simulink model "ssc_cvt_test_harness"  (R2025a)
settings: Solver=VariableStepAuto  StartTime=0.0  StopTime=200  RelTol=1e-3
undefined symbols (not defined in the file or in its folder): HMPST
libraries: fl_lib x7, nesl_utility x5, sm_wheel_loader_lib x3, sdl_lib x2, simulink x1
Description:
  | CVT Test Harness
  | Copyright 2024-2025 The MathWorks, Inc.
settings Model: Creator=smiller  LastModifiedBy=smiller
settings SolverCC: MaxConsecutiveMinStep=5
settings SimscapeCC: SimscapeLogType=all

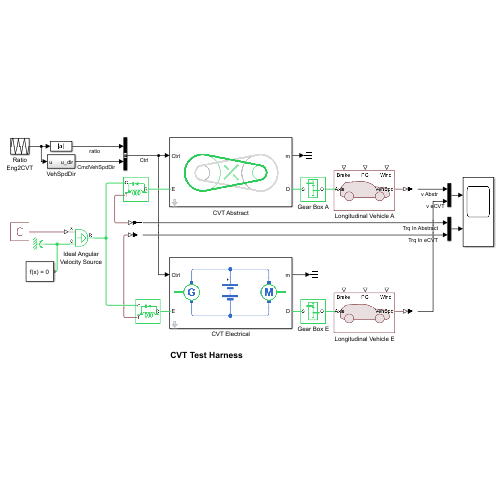
[thumbnail: Simulink's stored preview of the top-level diagram]
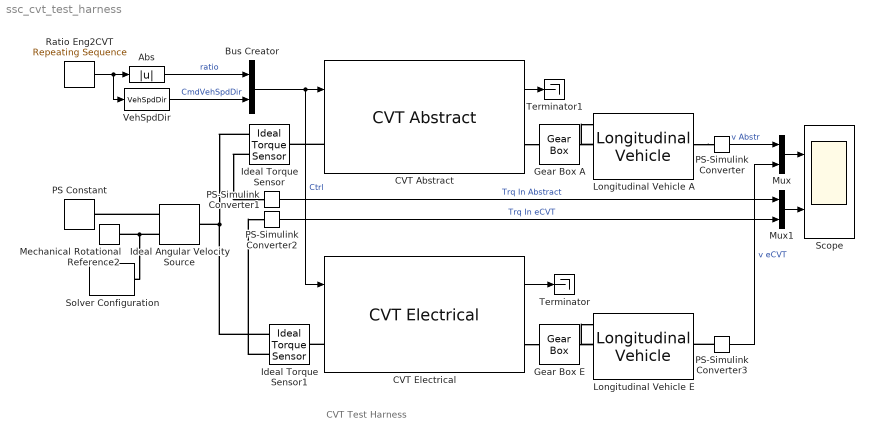
== system ssc_cvt_test_harness ==
  note: CVT Test Harness
  Abs : Abs  ZeroCross=off  SaturateOnIntegerOverflow=off
  Bus Creator : BusCreator  Inputs=2
  CVT Abstract : sm_wheel_loader_lib/CVT Abstract  dShaftE=HMPST.AbstractCVT.dInput  dShaftD=HMPST.AbstractCVT.dOutput  k=HMPST.AbstractCVT.kCompliance  d=HMPST.AbstractCVT.dCompliance
  CVT Electrical : sm_wheel_loader_lib/CVT Electrical  VariantControl=Electrical
  Gear Box A : fl_lib/Mechanical/Mechanisms/Gear Box  ratio=10  t_in_specify=off  t_in_priority=None  t_in=0 N*m  t_in_nominal_specify=off  t_in_nominal_value=1  t_in_nominal_unit=N*m  t_out_specify=off  t_out_priority=None  t_out=0 N*m  t_out_nominal_specify=off  t_out_nominal_value=1  t_out_nominal_unit=N*m
  Gear Box E : fl_lib/Mechanical/Mechanisms/Gear Box  ratio=10  t_in_specify=off  t_in_priority=None  t_in=0 N*m  t_in_nominal_specify=off  t_in_nominal_value=1  t_in_nominal_unit=N*m  t_out_specify=off  t_out_priority=None  t_out=0 N*m  t_out_nominal_specify=off  t_out_nominal_value=1  t_out_nominal_unit=N*m
  Ideal Angular Velocity Source : fl_lib/Mechanical/Mechanical Sources/Ideal Angular Velocity Source
  Ideal Torque Sensor : fl_lib/Mechanical/Mechanical Sensors/Ideal Torque Sensor
  Ideal Torque Sensor1 : fl_lib/Mechanical/Mechanical Sensors/Ideal Torque Sensor
  Longitudinal Vehicle A : sdl_lib/Tires & Vehicles/Longitudinal Vehicle  vehParamType=sdl.enum.VehicleParameterizationType.Regular  M_vehicle=3638 kg  R_tireroll=0.3 m  C_tireroll=0.0136  C_airdrag=0.31  A_front=2.3 m^2  A_rl=120 N  B_rl=1.8 N*s/m  C_rl=0.389 N*s^2/m^2  g=9.81 m/s^2  V_1=0.3 m/s  w_1=0.01 rad/s  ShowBrakeIn=true  ShowSlopeIn=true  SlopeInputType=sdl.enum.VehicleLongitudinalRoadSlopeInputType.GradePercent  ShowWindIn=true  ShowGOut=false  air_density=1.184 kg/m^3  V_x_specify=off  V_x_priority=High  V_x=0 m/s  V_x_nominal_specify=off  V_x_nominal_value=1  V_x_nominal_unit=m/s  trq_specify=off  trq_priority=None  trq=0 N*m  trq_nominal_specify=off  trq_nominal_value=1  trq_nominal_unit=N*m  w_specify=off  w_priority=None  w=0 rad/s  w_nominal_specify=off  w_nominal_value=1  w_nominal_unit=rad/s
      settings: InternalSimscapePortConfiguration="{\"Bottom\":[],\"Left\":[{\"id\":\"Axle\",\"label\":\"Axle\",\"type\":\"foundation.mechanical.rotational.rotational\"}],\"Right\":[{\"id\":\"v_out\",\"label\":\"VehSpd\",\"type\":\"output\"}],\"Top\":[{\"id\":\"brkF\",\"label\":\"Brake\",\"type\":\"input\"},{\"id\":\"grade_pct\",\"label\":\"PG\",\"type\":\"input\"},{\"id\":\"V_wind\",\"label\":\"Wind\",\"type\":\"input\"}]}"
  Longitudinal Vehicle E : sdl_lib/Tires & Vehicles/Longitudinal Vehicle  vehParamType=sdl.enum.VehicleParameterizationType.Regular  M_vehicle=3638 kg  R_tireroll=0.3 m  C_tireroll=0.0136  C_airdrag=0.31  A_front=2.3 m^2  A_rl=120 N  B_rl=1.8 N*s/m  C_rl=0.389 N*s^2/m^2  g=9.81 m/s^2  V_1=0.3 m/s  w_1=0.01 rad/s  ShowBrakeIn=true  ShowSlopeIn=true  SlopeInputType=sdl.enum.VehicleLongitudinalRoadSlopeInputType.GradePercent  ShowWindIn=true  ShowGOut=false  air_density=1.184 kg/m^3  V_x_specify=off  V_x_priority=High  V_x=0 m/s  V_x_nominal_specify=off  V_x_nominal_value=1  V_x_nominal_unit=m/s  trq_specify=off  trq_priority=None  trq=0 N*m  trq_nominal_specify=off  trq_nominal_value=1  trq_nominal_unit=N*m  w_specify=off  w_priority=None  w=0 rad/s  w_nominal_specify=off  w_nominal_value=1  w_nominal_unit=rad/s
      settings: InternalSimscapePortConfiguration="{\"Bottom\":[],\"Left\":[{\"id\":\"Axle\",\"label\":\"Axle\",\"type\":\"foundation.mechanical.rotational.rotational\"}],\"Right\":[{\"id\":\"v_out\",\"label\":\"VehSpd\",\"type\":\"output\"}],\"Top\":[{\"id\":\"brkF\",\"label\":\"Brake\",\"type\":\"input\"},{\"id\":\"grade_pct\",\"label\":\"PG\",\"type\":\"input\"},{\"id\":\"V_wind\",\"label\":\"Wind\",\"type\":\"input\"}]}"
  Mechanical Rotational Reference2 : fl_lib/Mechanical/Rotational Elements/Mechanical Rotational Reference
  Mux : Mux  Inputs=2
  Mux1 : Mux  Inputs=2
  PS Constant : fl_lib/Physical Signals/Sources/PS Constant  constant=2200 rpm
  PS-Simulink Converter{,1..3} (4 alike) : nesl_utility/PS-Simulink Converter  PhysicalDomain=network_engine_domain  SubClassName=ps_output  LeftPortType=input  RightPortType=output  PseudoPeriodic=off  Frequencies=[]  VectorFormat=inherit  Unit=inherit  AffineConversion=off
  Ratio Eng2CVT : simulink/Sources/Repeating Sequence  rep_seq_t=[0 5 95 105 195 200 205 295 305 395 400]/2  rep_seq_y=[0 0 2.1 2.1 0 0 0 -2.1 -2.1 0 0]
  Scope : Scope  NumInputPorts=2
      settings: ActiveDisplayYMinimum=-18.16022  ActiveDisplayYMaximum=18.16014
  Solver Configuration : nesl_utility/Solver Configuration  PhysicalDomain=network_engine_domain  SubClassName=solver  LeftPortType=input  RightPortType=generic  Tones=[]  Harmonics=[]  SimulateNoise=off  Profile=off  UseLocalSampling=off  EnableSwitchedLinearOptims=on  FrequencyDomain=off  UseCCode=off  RelTol=0.001  AbsTol=0.001  MinStep=1e-09  ToWorkspace=off  RevertToSquareIcSolve=off  NumHomotopyIterations=100  PhasorMode=off  PhasorModeNumHarmonics=1  ConsistencySolver=NEWTON_XTOL_AFTER_FTOL  IndexReductionMethod=DerivativeReplacement  DoDC=off  ResidualTolerance=1e-09  ConsistencyTolSource=GLOBAL  ConsistencyAbsTol=0.001  ConsistencyRelTol=0.001  ConsistencyTolFactor=0.001  UseLocalSolver=off  LocalSolverChoice=NE_BACKWARD_EULER_ADVANCER  ResolveIndetEquations=on  FunctionEvalNumThread=1  LocalSolverSampleTime=0.001  DoFixedCost=off  MaxNonlinIter=3  MaxModeIter=2  ComputeImpulses=off  ImpulseIterations=2  LinearAlgebra=auto  LinearAlgebraNumThread=0  EquationFormulation=NE_TIME_EF  DelaysMemoryBudget=1024  AutomaticFiltering=on  FilteringTimeConstant=0.001  PartitionStorageMethod=AS_NEEDED  PartitionMemoryBudget=1024  PartitionMethod=ROBUST  MultibodyUseLocalSolver=off  MultibodyLocalSolverChoice=ODE1  MultibodyLocalSolverSampleTime=0.001
  Terminator : Terminator
  Terminator1 : Terminator
  VehSpdDir : sm_wheel_loader_lib/Controller/Desired Ratio Calc/VehSpdDir  SystemSampleTime=-1  VariantActivationTime=update diagram  EmptyChoice=off  PassThrough=off  PassThroughVariantControl=(default)  EmptyChoiceVariantControl=(default)  AllowFlexibleInterface=on  Latency=0  AutoFrameSizeCalculation=off
  wires:
  PS-Simulink Converter/1 -> Mux/1  "v Abstr"
  Abs/1 -> Bus Creator/1  "ratio"
  Ratio Eng2CVT/1 -> Abs/1, VehSpdDir/1
  VehSpdDir/1 -> Bus Creator/2  "CmdVehSpdDir"
  Bus Creator/1 -> CVT Abstract/1, CVT Electrical/1  "Ctrl"
  PS-Simulink Converter3/1 -> Mux/2  "v eCVT"
  Mux/1 -> Scope/1
  Mux1/1 -> Scope/2
  PS-Simulink Converter1/1 -> Mux1/1  "Trq In Abstract"
  PS-Simulink Converter2/1 -> Mux1/2  "Trq In eCVT"
  CVT Electrical/1 -> Terminator/1
  CVT Abstract/1 -> Terminator1/1
  connections:
  Ideal Angular Velocity Source/RConn2 -- Mechanical Rotational Reference2/LConn1 -- Solver Configuration/RConn1
  Ideal Angular Velocity Source/RConn1 -- PS Constant/RConn1
  Longitudinal Vehicle A/RConn1 -- PS-Simulink Converter/LConn1
  Gear Box A/RConn1 -- Longitudinal Vehicle A/LConn1
  Ideal Torque Sensor/RConn1 -- Ideal Torque Sensor1/RConn1 -- Ideal Angular Velocity Source/LConn1
  CVT Abstract/LConn1 -- Ideal Torque Sensor/LConn1
  Ideal Torque Sensor/RConn2 -- PS-Simulink Converter1/LConn1
  CVT Electrical/LConn1 -- Ideal Torque Sensor1/LConn1
  Ideal Torque Sensor1/RConn2 -- PS-Simulink Converter2/LConn1
  CVT Electrical/RConn1 -- Gear Box E/LConn1
  PS-Simulink Converter3/LConn1 -- Longitudinal Vehicle E/RConn1
  CVT Abstract/RConn1 -- Gear Box A/LConn1
  Gear Box E/RConn1 -- Longitudinal Vehicle E/LConn1
